simulink model "SVPWM"  (R2021a)
settings: Solver=VariableStepAuto  StartTime=0.0  StopTime=0.1  FixedStep=10e-5  RelTol=1e-6
InitFcn:
  | cd 'F:\Learning\Power\FOC';
  | run('Params.m')
values from neighbouring files (symbols this model uses):
  Ts = 1/fs    (= 5e-05)    [Params.m]
  V_DC = 12    [Params.m]
undefined symbols (not defined in the file or in its folder): Down, Up
libraries: eePwmGenerator x3
settings Model: Creator=DEEL  LastModifiedBy=DEEL
settings SolverCC: ZeroCrossControl=DisableAll
settings DataIOCC: SaveOutput=off  SaveTime=off
settings OptimizationCC: DefaultParameterBehavior=Inlined  EnhancedBackFolding=on  PassReuseOutputArgsAs=Individual arguments  ZeroExternalMemoryAtStartup=off  ZeroInternalMemoryAtStartup=off  OptimizeBlockOrder=speed  DifferentSizesBufferReuse=on  OptimizationCustomize=off  EfficientTunableParamExpr=on
settings DebuggingCC: ParameterTunabilityLossMsg=error
settings SFSimCC: MATLABDynamicMemAlloc=off
settings RTWCC: SystemTargetFile=ert.tlc  TemplateMakefile=ert_default_tmf
settings CodeAppCC: ForceParamTrailComments=on  IgnoreCustomStorageClasses=off  OperatorAnnotations=on  SimulinkDataObjDesc=on  SFDataObjDesc=on  InsertBlockDesc=on
settings ERTTargetCC: TargetLangStandard=C99 (ISO)  GenerateSampleERTMain=on  InlinedParameterPlacement=NonHierarchical  RTWCAPISignals=on  RTWCAPIParams=on  ERTCustomFileTemplate=example_file_process.tlc

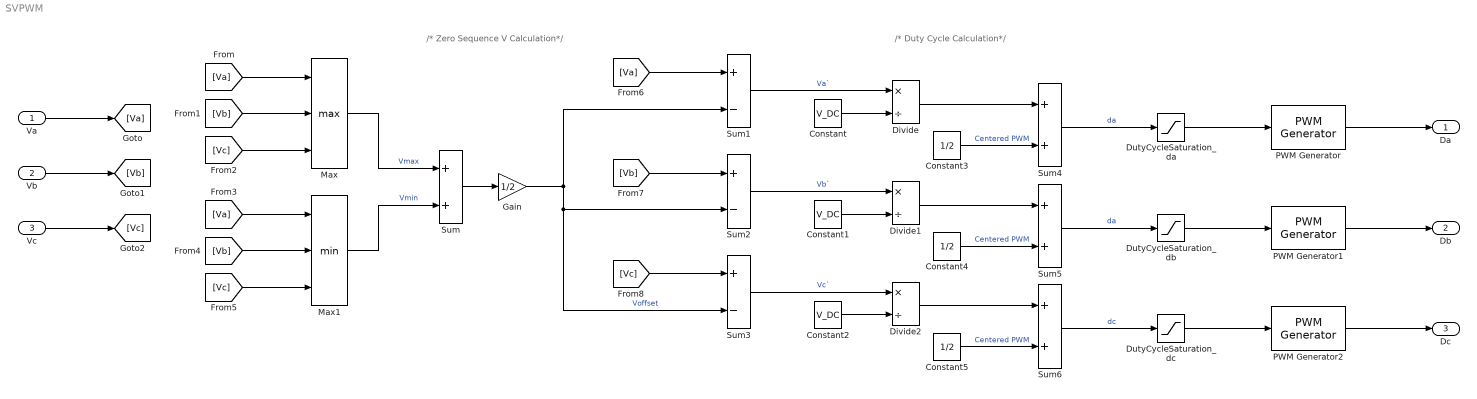
== system SVPWM ==
  note: /* Duty Cycle Calculation*/
  note: /* Zero Sequence V Calculation*/
  Va : Inport  OutDataTypeStr=double  PortDimensions=1  SampleTime=0
  Vb : Inport  Port=2  OutDataTypeStr=double  PortDimensions=1  SampleTime=0
  Vc : Inport  Port=3  OutDataTypeStr=double  PortDimensions=1  SampleTime=0
  Constant : Constant  Value=V_DC
  Constant1 : Constant  Value=V_DC
  Constant2 : Constant  Value=V_DC
  Constant3 : Constant  Value=1/2
  Constant4 : Constant  Value=1/2
  Constant5 : Constant  Value=1/2
  Divide : Product  Inputs=*/
  Divide1 : Product  Inputs=*/
  Divide2 : Product  Inputs=*/
  DutyCycleSaturation_da : Saturate  UpperLimit=1  LowerLimit=0
  DutyCycleSaturation_db : Saturate  UpperLimit=1  LowerLimit=0
  DutyCycleSaturation_dc : Saturate  UpperLimit=1  LowerLimit=0
  Gain : Gain  Gain=1/2
  Max : MinMax  Function=max  Inputs=3
  Max1 : MinMax  Inputs=3
  PWM Generator : eePwmGenerator/PWM Generator  CarrCount=Up-Down  Tper=Ts  Ts=Ts/100
  PWM Generator1 : eePwmGenerator/PWM Generator  CarrCount=Up-Down  Tper=Ts  Ts=Ts/100
  PWM Generator2 : eePwmGenerator/PWM Generator  CarrCount=Up-Down  Tper=Ts  Ts=Ts/100
  Sum{,4..6} (4 alike) : Sum
  Sum1 : Sum  Inputs=+-
  Sum2 : Sum  Inputs=+-
  Sum3 : Sum  Inputs=+-
  Da : Outport  OutDataTypeStr=boolean  PortDimensions=1  SampleTime=[4.9999999999999998e-07,0]
  Db : Outport  Port=2  OutDataTypeStr=boolean  PortDimensions=1  SampleTime=[4.9999999999999998e-07,0]
  Dc : Outport  Port=3  OutDataTypeStr=boolean  PortDimensions=1  SampleTime=[4.9999999999999998e-07,0]
  wires:
  Max/1 -> Sum/1  "Vmax"
  Max1/1 -> Sum/2  "Vmin"
  Sum/1 -> Gain/1
  Gain/1 -> Sum2/2, Sum3/2, Sum1/2  "Voffset"
  Va/1 -> [Va]
  Vb/1 -> [Vb]
  Vc/1 -> [Vc]
  [Va] -> Max/1
  [Vb] -> Max/2
  [Vc] -> Max/3
  [Va] -> Max1/1
  [Vb] -> Max1/2
  [Vc] -> Max1/3
  [Va] -> Sum1/1
  [Vb] -> Sum2/1
  [Vc] -> Sum3/1
  Sum1/1 -> Divide/1  "Va`"
  Constant/1 -> Divide/2
  Constant1/1 -> Divide1/2
  Constant2/1 -> Divide2/2
  Sum2/1 -> Divide1/1  "Vb`"
  Sum3/1 -> Divide2/1  "Vc`"
  Constant3/1 -> Sum4/2  "Centered PWM"
  Divide/1 -> Sum4/1
  Divide1/1 -> Sum5/1
  Constant4/1 -> Sum5/2  "Centered PWM"
  Constant5/1 -> Sum6/2  "Centered PWM"
  Divide2/1 -> Sum6/1
  Sum4/1 -> DutyCycleSaturation_da/1  "da"
  Sum5/1 -> DutyCycleSaturation_db/1  "da"
  Sum6/1 -> DutyCycleSaturation_dc/1  "dc"
  DutyCycleSaturation_da/1 -> PWM Generator/1
  DutyCycleSaturation_db/1 -> PWM Generator1/1
  DutyCycleSaturation_dc/1 -> PWM Generator2/1
  PWM Generator/1 -> Da/1
  PWM Generator2/1 -> Dc/1
  PWM Generator1/1 -> Db/1
